simulink model "T12_Sim_BPSK_3"  (R2015a)
settings: Solver=ode45  StartTime=0.0  StopTime=50  RelTol=1e-3
libraries: commdigbbndpm3 x2, commchan3 x1, commrandsrc2 x1
settings Model: Creator=User  LastModifiedBy=User

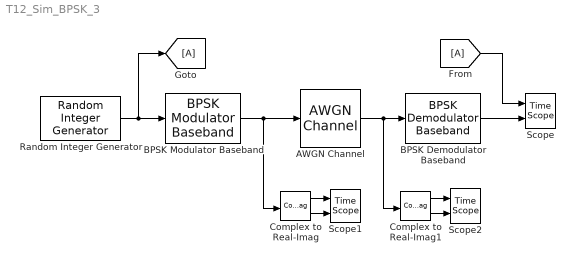
== system T12_Sim_BPSK_3 ==
  AWGN Channel : commchan3/AWGN Channel  InputProcessing=Columns as channels (frame based)  seed=67  noiseMode="Signal to noise ratio  (Eb/No)"  EbNodB=0  EsNodB=4  SNRdB=10  bitsPerSym=1  Ps=1  Tsym=1  variance=1
  BPSK Demodulator Baseband : commdigbbndpm3/BPSK Demodulator Baseband  Ph=0  DecType=Hard decision  VarSource=Dialog  Variance=1  outDtype=Inherit via internal rule  derotateFactorWordLen=16
  BPSK Modulator Baseband : commdigbbndpm3/BPSK Modulator Baseband  Ph=0  outDtype=double  outWordLen=16  outUDDataType=sfix(16)  outFracLenMode=Best precision  outFracLen=15
  Complex to Real-Imag : ComplexToRealImag
  Complex to Real-Imag1 : ComplexToRealImag
  Random Integer Generator : commrandsrc2/Random Integer Generator  mul=2  seed=37  Ts=1  frameBased=off  sampPerFrame=1000  orient=off  outDataType=boolean
  Scope : TimeScope  NumInputPorts=2
  Scope1 : TimeScope  NumInputPorts=2
  Scope2 : TimeScope  NumInputPorts=2
  wires:
  Random Integer Generator/1 -> [A], BPSK Modulator Baseband/1
  BPSK Modulator Baseband/1 -> Complex to Real-Imag/1, AWGN Channel/1
  AWGN Channel/1 -> Complex to Real-Imag1/1, BPSK Demodulator Baseband/1
  BPSK Demodulator Baseband/1 -> Scope/2
  [A] -> Scope/1
  Complex to Real-Imag/1 -> Scope1/1
  Complex to Real-Imag/2 -> Scope1/2
  Complex to Real-Imag1/1 -> Scope2/1
  Complex to Real-Imag1/2 -> Scope2/2
